simulink model "mod_psk8"  (R2024b)
settings: Solver=FixedStepDiscrete  StartTime=0.0  StopTime=1  FixedStep=3.1250000000000001e-05  RelTol=1e-3
model workspace (MAT data in the model file):
  M = 8
  Ts = 0.001
  decalage = 0
  df_ol = 1
  fc = 4000
  fs = 32000
  gain_ech = 1.00703119427
  graine = 7
  h_rx = [8.56459526083e-05 0.000117681393507 0.000148802662364 0.000178447986179 0.000206066607265 0.000231128526307 0.000253134118628 0.000271623456863 0.000286185174424 0.000296464708155 0.000302171765366 0.00030308687003 ... (353 elements, 1x353)]
  h_tx = [0.00274067048347 0.00376580459222 0.00476168519565 0.00571033555773 0.00659413143249 0.00739611284184 0.0081002917961 0.00869195061961 0.00915792558158 0.00948687066094 0.00966949649171 0.00969877984097 ... (353 elements, 1x353)]
  ordre = 8
  phi_ol = 0.7
  points = [0.923879532511+0.382683432365i 0.382683432365+0.923879532511i -0.382683432365+0.923879532511i -0.923879532511+0.382683432365i -0.923879532511-0.382683432365i -0.382683432365-0.923879532511i 0.382683432365-0.923879532511i 0.923879532511-0.382683432365i]
  ptsI = [0.923879532511 0.382683432365 -0.382683432365 -0.923879532511 -0.923879532511 -0.382683432365 0.382683432365 0.923879532511]
  ptsQ = [0.382683432365 0.923879532511 0.923879532511 0.382683432365 -0.382683432365 -0.923879532511 -0.923879532511 -0.382683432365]
  sigma2 = 0
  sps = 32
  w_boucle = 0.000490873852123
settings Model: Creator=runner  LastModifiedBy=runner

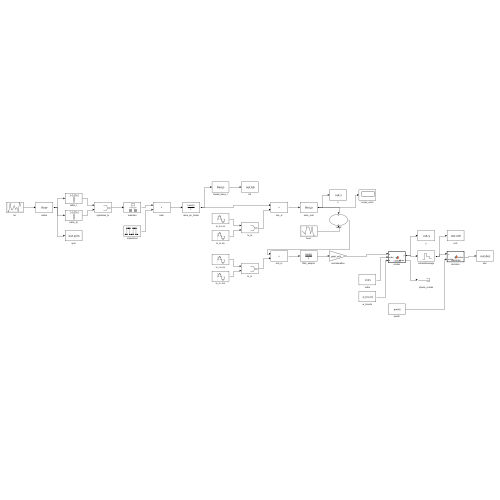
[thumbnail: Simulink's stored preview of the top-level diagram]
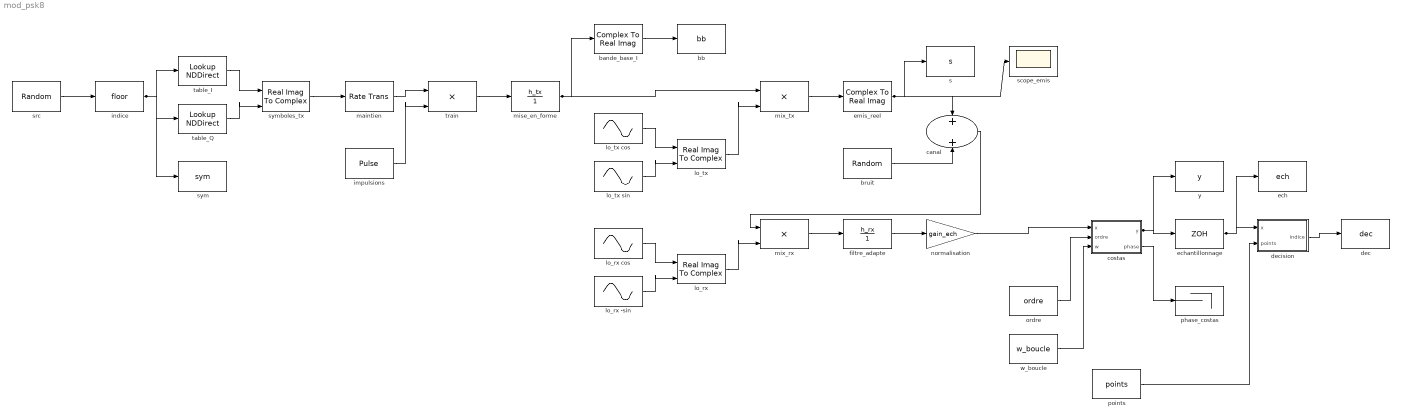
== system mod_psk8 ==
  bande_base_I : ComplexToRealImag  Output=Real
  bb : ToWorkspace  VariableName=bb  SampleTime=-1
  bruit : RandomNumber  Variance=sigma2  Seed=1  SampleTime=1/fs
  canal : Sum
  costas : MATLAB Function  TreatAsAtomicUnit=on
  dec : ToWorkspace  VariableName=dec  SampleTime=-1
  decision : MATLAB Function  TreatAsAtomicUnit=on
  ech : ToWorkspace  VariableName=ech  SampleTime=-1
  echantillonnage : ZeroOrderHold  SampleTime=[Ts, decalage]
  emis_reel : ComplexToRealImag  Output=Real
  filtre_adapte : DiscreteFilter  Numerator=h_rx  Denominator=1
  impulsions : DiscretePulseGenerator  Period=sps  SampleTime=1/fs
  indice : Rounding
  lo_rx : RealImagToComplex
  lo_rx -sin : Sin  Amplitude=-2  Frequency=2*pi*(fc+df_ol)  Phase=phi_ol  SampleTime=1/fs
  lo_rx cos : Sin  Amplitude=2  Frequency=2*pi*(fc+df_ol)  Phase=phi_ol+pi/2  SampleTime=1/fs
  lo_tx : RealImagToComplex
  lo_tx cos : Sin  Frequency=2*pi*fc  Phase=pi/2  SampleTime=1/fs
  lo_tx sin : Sin  Frequency=2*pi*fc  SampleTime=1/fs
  maintien : RateTransition  OutPortSampleTime=1/fs
  mise_en_forme : DiscreteFilter  Numerator=h_tx  Denominator=1
  mix_rx : Product
  mix_tx : Product
  normalisation : Gain  Gain=gain_ech
  ordre : Constant  Value=ordre
  phase_costas : Terminator
  points : Constant  Value=points
  s : ToWorkspace  VariableName=s  SampleTime=-1
  scope_emis : Scope
  src : UniformRandomNumber  Minimum=0  Maximum=M  Seed=graine  SampleTime=Ts
  sym : ToWorkspace  VariableName=sym  SampleTime=-1
  symboles_tx : RealImagToComplex
  table_I : LookupNDDirect  NumberOfTableDimensions=1  Table=ptsI
  table_Q : LookupNDDirect  NumberOfTableDimensions=1  Table=ptsQ
  train : Product
  w_boucle : Constant  Value=w_boucle
  y : ToWorkspace  VariableName=y  SampleTime=-1
  wires:
  src/1 -> indice/1
  indice/1 -> table_I/1, table_Q/1, sym/1
  table_I/1 -> symboles_tx/1
  table_Q/1 -> symboles_tx/2
  symboles_tx/1 -> maintien/1
  maintien/1 -> train/1
  impulsions/1 -> train/2
  train/1 -> mise_en_forme/1
  mise_en_forme/1 -> bande_base_I/1, mix_tx/1
  bande_base_I/1 -> bb/1
  lo_tx cos/1 -> lo_tx/1
  lo_tx sin/1 -> lo_tx/2
  lo_tx/1 -> mix_tx/2
  mix_tx/1 -> emis_reel/1
  emis_reel/1 -> canal/1, s/1, scope_emis/1
  bruit/1 -> canal/2
  lo_rx cos/1 -> lo_rx/1
  lo_rx -sin/1 -> lo_rx/2
  canal/1 -> mix_rx/1
  lo_rx/1 -> mix_rx/2
  mix_rx/1 -> filtre_adapte/1
  filtre_adapte/1 -> normalisation/1
  normalisation/1 -> costas/1(x)
  ordre/1 -> costas/2(ordre)
  w_boucle/1 -> costas/3(w)
  costas/1(y) -> y/1, echantillonnage/1
  costas/2(phase) -> phase_costas/1
  echantillonnage/1 -> ech/1, decision/1(x)
  points/1 -> decision/2(points)
  decision/1(indice) -> dec/1

== matlab function mod_psk8/decision ==
  data: x input; indice output; points input
function indice = decision(x, points)
% decision au plus proche voisin, comme le bloc Constellation Decoder de GNU Radio
[~, k] = min(abs(x - points));
indice = k - 1;
end

== matlab function mod_psk8/costas ==
  data: x input; y output; ordre input; w input; phase output
function [y, phase] = costas(x, ordre, w)
% boucle de Costas, meme algorithme que le bloc Costas Loop de GNU Radio 3.10
persistent ph fr
if isempty(ph), ph = 0; fr = 0; end
z = sqrt(2) / 2; den = 1 + 2 * z * w + w * w; a = 4 * z * w / den; b = 4 * w * w / den;
y = x * exp(-1j * ph); r = real(y); q = imag(y); K = sqrt(2) - 1;
if ordre == 2
    e = r * q;
elseif ordre == 4
    e = sg(r) * q - sg(q) * r;
elseif abs(r) >= abs(q)
    e = sg(r) * q - K * sg(q) * r;
else
    e = K * sg(r) * q - sg(q) * r;
end
e = max(-1, min(1, e)); fr = fr + b * e; ph = ph + fr + a * e;
ph = mod(ph + pi, 2 * pi) - pi; fr = max(-1, min(1, fr)); phase = ph;
end
function s = sg(v)
if v > 0, s = 1; else, s = -1; end
end
